simulink model "HVAC_Sim"  (R2026a)
settings: Solver=ode45  StopTime=T_END  MaxStep=Ts
values from neighbouring files (symbols this model uses):
  CTRL = d.ctrl    [analyze_results.m]    (also in build_hvac_model.m = 2; hw_run_control.m = 2)
  K = 1.41    [hvac_identified.mat]    (also in hvac_params.m = S.K; identify_model.m = p(1))
  L = 0.187187657432    [hvac_identified.mat]    (also in hvac_params.m = max(L, Ts); identify_model.m = p(3))
  Ta = d.Ta_lat    [analyze_results.m]    (also in hvac_params.m = 24)
  tau = 19.6    [hvac_identified.mat]    (also in hvac_params.m = S.tau; identify_model.m = max(p(2), Ts))
  tau_s = 1.0    (= 1)    [hvac_params.m]
  Ts = 0.5    [hvac_params.m]
  U_MAX = 5.0    (= 5)    [hvac_params.m]
undefined symbols (not defined in the file or in its folder): FD, ONOFF, PI
libraries: slpidlib x1, simulink x1
settings Model: Creator=lenovo  LastModifiedBy=lenovo

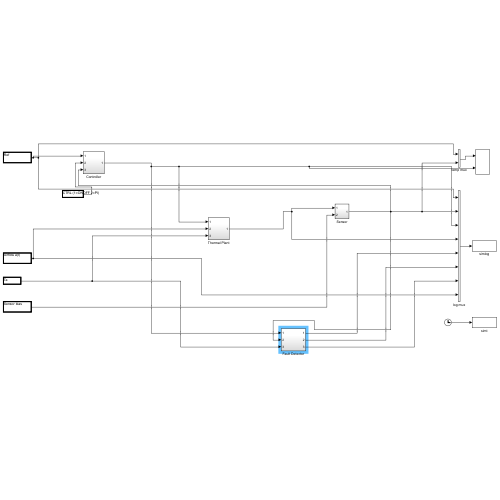
[thumbnail: Simulink's stored preview of the top-level diagram]
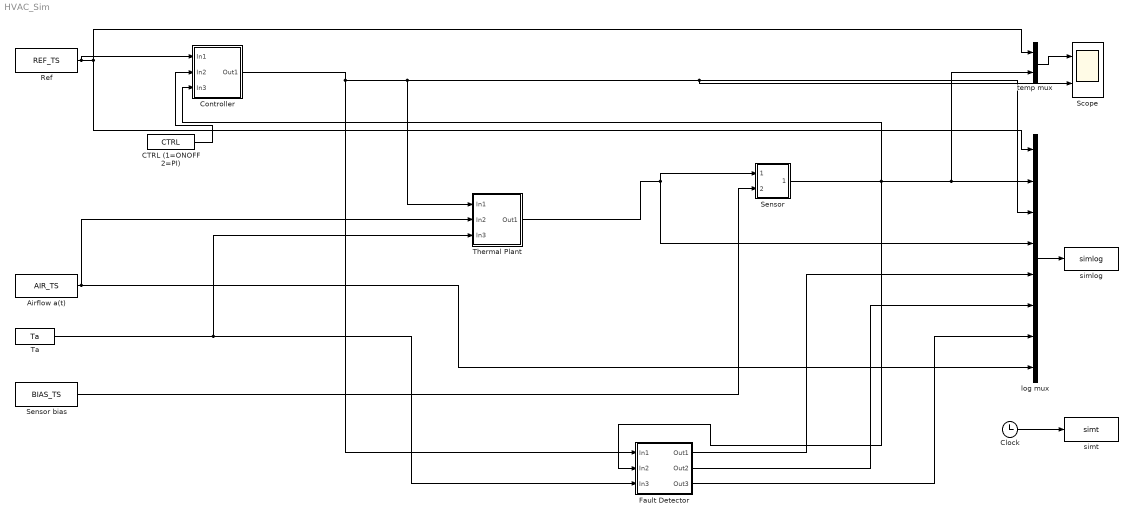
== system HVAC_Sim ==
  Airflow a(t) : FromWorkspace  VariableName=AIR_TS  SampleTime=Ts  Interpolate=off  OutputAfterFinalValue=Holding final value
  CTRL (1=ONOFF 2=PI) : Constant  Value=CTRL
  Clock : Clock
  Controller : Subsystem
  Fault Detector : Subsystem
  Ref : FromWorkspace  VariableName=REF_TS  SampleTime=Ts  Interpolate=off  OutputAfterFinalValue=Holding final value
  Scope : Scope  NumInputPorts=2
  Sensor : Subsystem
  Sensor bias : FromWorkspace  VariableName=BIAS_TS  SampleTime=Ts  Interpolate=off  OutputAfterFinalValue=Holding final value
  Ta : Constant  Value=Ta
  Thermal Plant : Subsystem
  log mux : Mux  Inputs=8
  simlog : ToWorkspace  VariableName=simlog  SampleTime=Ts
  simt : ToWorkspace  VariableName=simt  SampleTime=Ts
  temp mux : Mux  Inputs=2
  wires:
  Ref/1 -> log mux/1, temp mux/1, Controller/1(In1)
  Ta/1 -> Fault Detector/3(In3), Thermal Plant/3(In3)
  Airflow a(t)/1 -> Thermal Plant/2(In2), log mux/8
  log mux/1 -> simlog/1
  Clock/1 -> simt/1
  temp mux/1 -> Scope/1
  Thermal Plant/1(Out1) -> Sensor/1(In1), log mux/4
  Sensor/1(Out1) -> Fault Detector/2(In2), Controller/3(In3), log mux/2, temp mux/2
  Sensor bias/1 -> Sensor/2(In2)
  Controller/1(Out1) -> Fault Detector/1(In1), log mux/3, Scope/2, Thermal Plant/1(In1)
  CTRL (1=ONOFF 2=PI)/1 -> Controller/2(In2)
  Fault Detector/1(Out1) -> log mux/5
  Fault Detector/2(Out2) -> log mux/6
  Fault Detector/3(Out3) -> log mux/7

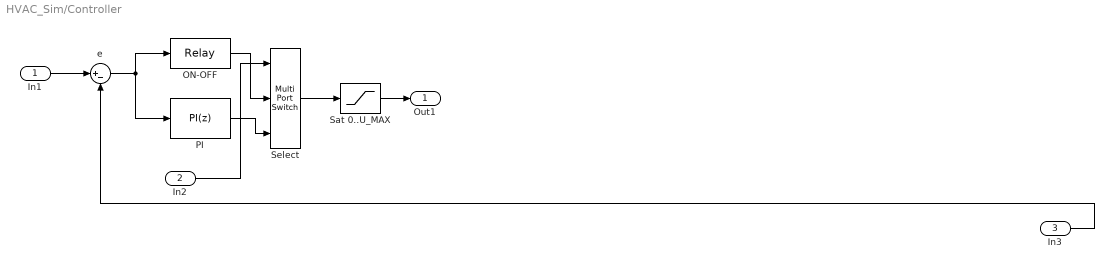
== system HVAC_Sim/Controller ==
  In1 : Inport
  In2 : Inport  Port=2
  In3 : Inport  Port=3
  ON-OFF : Relay  OnSwitchValue=ONOFF.H/2  OffSwitchValue=-ONOFF.H/2  OnOutputValue=ONOFF.U_ON
  PI : slpidlib/PID Controller  Controller=PI  Form=Parallel  TimeDomain=Discrete-time  UseExternalTs=off  SampleTime=Ts  IntegratorMethod=Forward Euler  FilterMethod=Forward Euler  ControllerParametersSource=internal  P=PI.Kp  I=PI.Ki  UseKiTs=off  D=0  UseExternalDerivativeSource=off  N=100  UseFilter=on  TunerSelectOption=Transfer Function Based (PID Tuner App)  InitialConditionSource=internal  InitialConditionForIntegrator=0  InitialConditionForFilter=0  DifferentiatorICPrevScaledInput=0  ExternalReset=none  TrackingMode=off  Kt=1  LimitOutput=on  SatLimitsSource=internal  UpperSaturationLimit=U_MAX  LowerSaturationLimit=0  LinearizeAsGain=off  AntiWindupMode=clamping  Kb=1  LimitIntegrator=off  UpperIntegratorSaturationLimit=inf  LowerIntegratorSaturationLimit=-inf  POutMin=[]  POutMax=[]  IOutMin=[]  IOutMax=[]  DOutMin=[]  DOutMax=[]  NOutMin=[]  NOutMax=[]  SumOutMin=[]  SumOutMax=[]  SaturationOutMin=[]  SaturationOutMax=[]  PParamMin=[]  PParamMax=[]  IParamMin=[]  IParamMax=[]  DParamMin=[]  DParamMax=[]  NParamMin=[]  NParamMax=[]  KbParamMin=[]  KbParamMax=[]  KtParamMin=[]  KtParamMax=[]  KbOutMin=[]  KbOutMax=[]  KtOutMin=[]  KtOutMax=[]  IntegratorOutMin=[]  IntegratorOutMax=[]  FilterOutMin=[]  FilterOutMax=[]  SumI1OutMin=[]  SumI1OutMax=[]  SumI2OutMin=[]  SumI2OutMax=[]  SumI3OutMin=[]  SumI3OutMax=[]  SumI4OutMin=[]  SumI4OutMax=[]  SumDOutMin=[]  SumDOutMax=[]  DifferentiatorOutMin=[]  DifferentiatorOutMax=[]  FilterDiffOutCoefMin=[]  FilterDiffOutCoefMax=[]  ReciprocalOutMin=[]  ReciprocalOutMax=[]  SumDenOutMin=[]  SumDenOutMax=[]  SumNumOutMin=[]  SumNumOutMax=[]  DivideOutMin=[]  DivideOutMax=[]  UdiffTsProdOutMin=[]  UdiffTsProdOutMax=[]  NTsProdOutMin=[]  NTsProdOutMax=[]  UintegralTsProdOutMin=[]  UintegralTsProdOutMax=[]  UngainTsProdOutMin=[]  UngainTsProdOutMax=[]  ClampingZeroOutDataTypeStr=Inherit: Inherit via back propagation  ClampingZeroOutMin=[]  ClampingZeroOutMax=[]  FilterDenConstantOutDataTypeStr=Inherit: Inherit via back propagation  FilterDenConstantOutMin=[]  FilterDenConstantOutMax=[]  PCopyOutDataTypeStr=Inherit: Inherit via back propagation  PCopyOutMin=[]  PCopyOutMax=[]  NCopyOutDataTypeStr=Inherit: Inherit via back propagation  NCopyOutMin=[]  NCopyOutMax=[]  IntegratorContinuousStateAttributes=''  IntegratorStateMustResolveToSignalObject=off  IntegratorRTWStateStorageClass=Auto  FilterContinuousStateAttributes=''  FilterStateMustResolveToSignalObject=off  FilterRTWStateStorageClass=Auto  ParallelPVariant=InternalParameters  IdealPVariant=Disabled  IVariant=InternalParameters  DVariant=Disabled  IntegratorVariant=Discrete  SatVariant=Enabled  AWVariant=DiscClampingParallel  PCopyVariant=Disabled  TRVariant=Disabled  FdbkBlocksVariant=Forward  IdealPFdbkVariant=Disabled  SatFdbkVariant=Disabled  DerivativeFilterVariant=Disabled  NVariant=Disabled  NCopyVariant=Disabled_SignalSpec  FilterICVariant=Disabled  IntegratorICVariant=InternalICs  ExternalResetVariant=Disabled  TRSumVariant=Passthrough  SumFdbkVariant=Disabled  SumVariant=Sum_PI  TsampFilterVariant=InternalTs  TsampNgainVariant=Passthrough  TsampIntegralVariant=Disabled_SignalSpec  ExternalSaturationOutDataTypeStr=Inherit: Same as second input  DerivativeSourceVariant=Disabled  PreIntVariant=InternalPreInt
      settings: LibrarySourceBlock=simulink/Discrete/Discrete PID Controller
  Sat 0..U_MAX : Saturate  UpperLimit=U_MAX  LowerLimit=0
  Select : MultiPortSwitch  Inputs=2  SaturateOnIntegerOverflow=off  InputSameDT=off
  e : Sum  Inputs=|+-
  Out1 : Outport
  wires:
  In1/1 -> e/1
  e/1 -> ON-OFF/1, PI/1
  PI/1 -> Select/3
  Select/1 -> Sat 0..U_MAX/1
  ON-OFF/1 -> Select/2
  In2/1 -> Select/1
  In3/1 -> e/2
  Sat 0..U_MAX/1 -> Out1/1

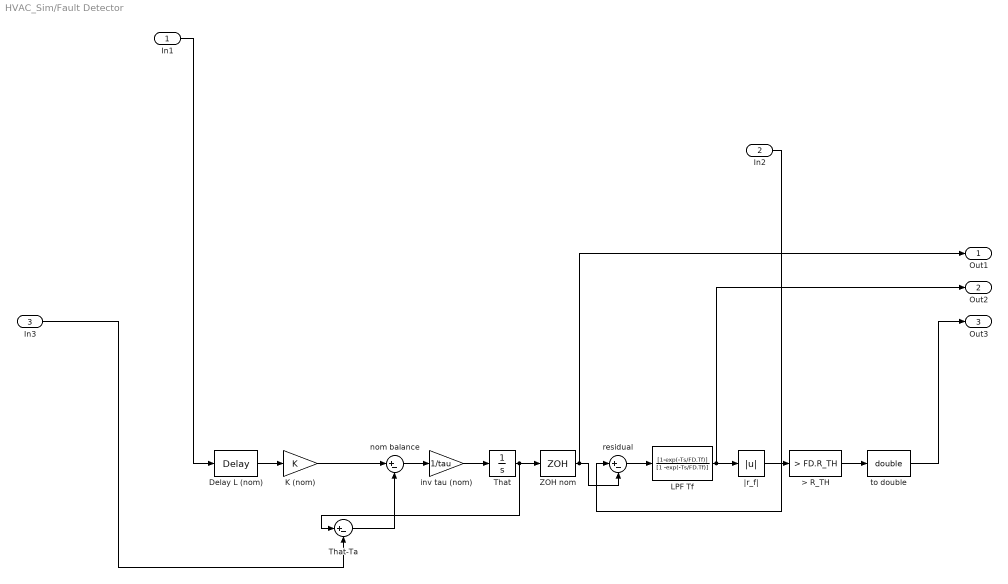
== system HVAC_Sim/Fault Detector ==
  In1 : Inport
  In2 : Inport  Port=2
  In3 : Inport  Port=3
  > R_TH : simulink/Logic and Bit Operations/Compare To Constant  relop=>  const=FD.R_TH  OutDataTypeStr=boolean
  Delay L (nom) : TransportDelay  DelayTime=L
  K (nom) : Gain  Gain=K
  LPF Tf : DiscreteTransferFcn  Numerator=[1-exp(-Ts/FD.Tf)]  Denominator=[1 -exp(-Ts/FD.Tf)]  SampleTime=Ts
  That : Integrator  InitialCondition=Ta
  That-Ta : Sum  Inputs=|+-
  ZOH nom : ZeroOrderHold  SampleTime=Ts
  inv tau (nom) : Gain  Gain=1/tau
  nom balance : Sum  Inputs=|+-
  residual : Sum  Inputs=|+-
  to double : DataTypeConversion  OutDataTypeStr=double  SaturateOnIntegerOverflow=off  RndMeth=Floor
  |r_f| : Abs  SaturateOnIntegerOverflow=off
  Out1 : Outport
  Out2 : Outport  Port=2
  Out3 : Outport  Port=3
  wires:
  That/1 -> That-Ta/1, ZOH nom/1
  inv tau (nom)/1 -> That/1
  That-Ta/1 -> nom balance/2
  nom balance/1 -> inv tau (nom)/1
  In2/1 -> residual/1
  |r_f|/1 -> > R_TH/1
  Delay L (nom)/1 -> K (nom)/1
  K (nom)/1 -> nom balance/1
  residual/1 -> LPF Tf/1
  ZOH nom/1 -> Out1/1, residual/2
  LPF Tf/1 -> Out2/1, |r_f|/1
  > R_TH/1 -> to double/1
  In3/1 -> That-Ta/2
  to double/1 -> Out3/1
  In1/1 -> Delay L (nom)/1

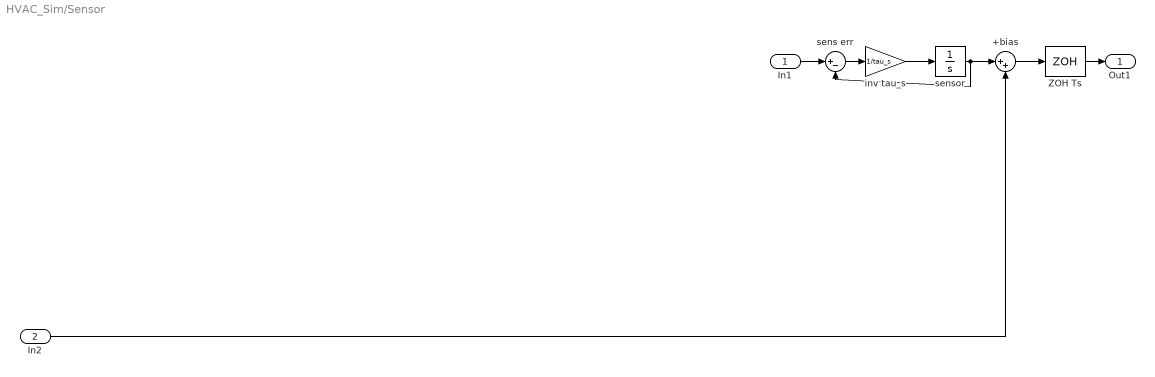
== system HVAC_Sim/Sensor ==
  In1 : Inport
  In2 : Inport  Port=2
  +bias : Sum  Inputs=|++
  ZOH Ts : ZeroOrderHold  SampleTime=Ts
  inv tau_s : Gain  Gain=1/tau_s
  sens err : Sum  Inputs=|+-
  sensor : Integrator  InitialCondition=Ta
  Out1 : Outport
  wires:
  sensor/1 -> sens err/2, +bias/1
  sens err/1 -> inv tau_s/1
  In1/1 -> sens err/1
  In2/1 -> +bias/2
  inv tau_s/1 -> sensor/1
  +bias/1 -> ZOH Ts/1
  ZOH Ts/1 -> Out1/1

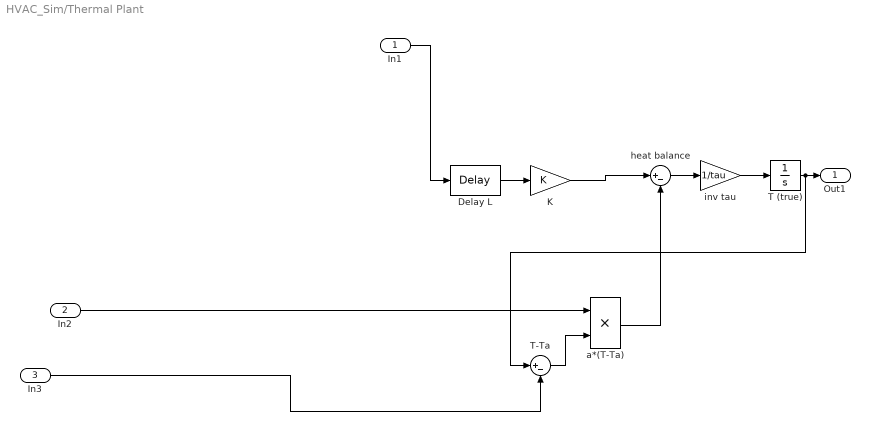
== system HVAC_Sim/Thermal Plant ==
  In1 : Inport
  In2 : Inport  Port=2
  In3 : Inport  Port=3
  Delay L : TransportDelay  DelayTime=L
  K : Gain  Gain=K
  T (true) : Integrator  InitialCondition=Ta
  T-Ta : Sum  Inputs=|+-
  a*(T-Ta) : Product
  heat balance : Sum  Inputs=|+-
  inv tau : Gain  Gain=1/tau
  Out1 : Outport
  wires:
  Delay L/1 -> K/1
  T (true)/1 -> T-Ta/1, Out1/1
  In1/1 -> Delay L/1
  a*(T-Ta)/1 -> heat balance/2
  T-Ta/1 -> a*(T-Ta)/2
  K/1 -> heat balance/1
  heat balance/1 -> inv tau/1
  inv tau/1 -> T (true)/1
  In3/1 -> T-Ta/2
  In2/1 -> a*(T-Ta)/1
